simulink model "Q4"  (R2023b)
settings: Solver=FixedStepAuto  StartTime=0.0  StopTime=10  FixedStep=0.1  RelTol=1e-3
settings Model: Creator=Arshia  LastModifiedBy=Arshia

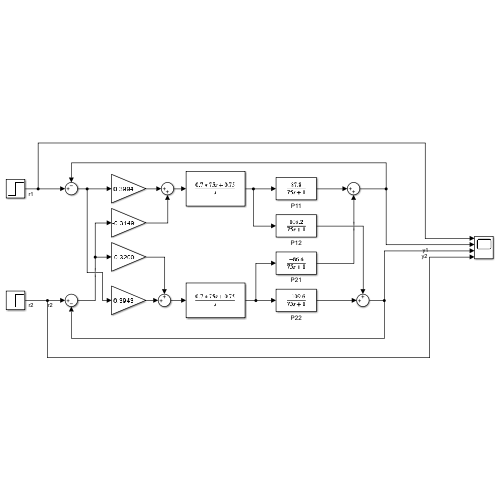
[thumbnail: Simulink's stored preview of the top-level diagram]
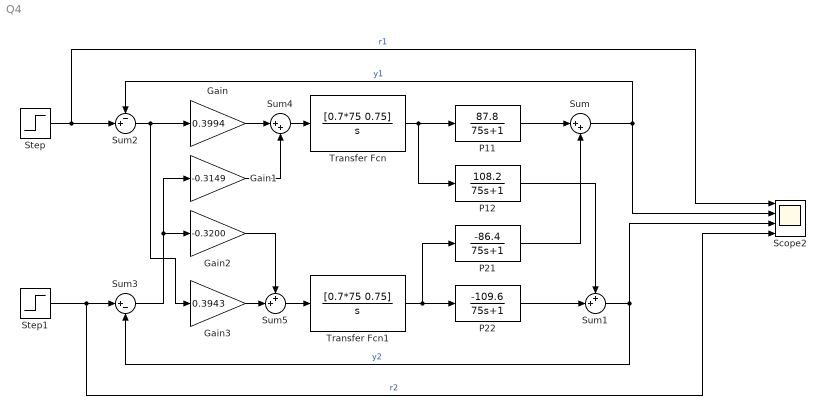
== system Q4 ==
  Gain : Gain  Gain=0.3994
  Gain1 : Gain  Gain=-0.3149
  Gain2 : Gain  Gain=-0.3200
  Gain3 : Gain  Gain=0.3943
  P11 : TransferFcn  Numerator=[87.8]  Denominator=[75 1]
  P12 : TransferFcn  Numerator=[108.2]  Denominator=[75 1]
  P21 : TransferFcn  Numerator=[-86.4]  Denominator=[75 1]
  P22 : TransferFcn  Numerator=[-109.6]  Denominator=[75 1]
  Scope2 : Scope  NumInputPorts=4
  Step : Step  Time=0  SampleTime=0
  Step1 : Step  Time=0  SampleTime=0
  Sum : Sum  Inputs=|++
  Sum1 : Sum  Inputs=++|
  Sum2 : Sum  Inputs=-+|
  Sum3 : Sum  Inputs=|+-
  Sum4 : Sum  Inputs=|++
  Sum5 : Sum  Inputs=++|
  Transfer Fcn : TransferFcn  Numerator=[0.7*75 0.75]  Denominator=[1 0]
  Transfer Fcn1 : TransferFcn  Numerator=[0.7*75 0.75]  Denominator=[1 0]
  wires:
  P11/1 -> Sum/1
  P21/1 -> Sum/2
  P12/1 -> Sum1/1
  P22/1 -> Sum1/2
  Sum/1 -> Sum2/1, Scope2/2  "y1"
  Sum1/1 -> Sum3/2, Scope2/3  "y2"
  Step/1 -> Sum2/2, Scope2/1  "r1"
  Step1/1 -> Sum3/1, Scope2/4  "r2"
  Transfer Fcn/1 -> P11/1, P12/1
  Transfer Fcn1/1 -> P21/1, P22/1
  Sum2/1 -> Gain3/1, Gain/1
  Sum3/1 -> Gain2/1, Gain1/1
  Gain/1 -> Sum4/1
  Gain1/1 -> Sum4/2
  Sum4/1 -> Transfer Fcn/1
  Gain2/1 -> Sum5/1
  Gain3/1 -> Sum5/2
  Sum5/1 -> Transfer Fcn1/1
